simulink library "ConverterLibrary"  (R2026a)
settings: Solver=VariableStepAuto
undefined symbols (not defined in the file or in its folder): DiscIntNeverNeededParam, dspblkCoreblockFVToolHelper, gcbh, gridInverter
libraries: fl_lib x240, nesl_utility x221, ee_lib x208, slpidlib x28, eeGeneralControl x12, simulink x9, eeTransforms x4, simulink_extras x1, eePowerMeasurement x1
(part 25 of 30)

== system ConverterLibrary/Power Converter Plant/Soft-Switching Converters/LLC Converter/LLC Primary Inverter and Resonant Tank/LLC Detailed Model/Inverter/Primary Inverter ==
  G1 : Inport
  G2 : Inport  Port=2
  G3 : Inport  Port=3
  G4 : Inport  Port=4
  Full Bridge with Thermal : Subsystem  VariantControl=FullBridgewithThermal
      settings: PortSchema="{\"entries\":[{\"content\":{\"sides\":[{\"content\":{\"connectorIds\":[\"LConn1\",\"LConn2\"]},\"type\":\"ConnectorPlacement.EquallySpacedRectSide\",\"uuid\":\"27c41940-d662-4779-afdd-48b642f77411\"},{\"content\":{\"connectorIds\":[\"RConn1\",\"RConn2\"],\"side\":\"RIGHT\"},\"type\":\"ConnectorPlacement.EquallySpacedRectSide\",\"uuid\":\"b0072b01-add1-4b0f-b94e-e1b6c9886b0e\"},{\"content\":{\"connectorIds\":[\"In1\",\"In2\",\"In3\",\"In4\"],\"side\":\"TOP\"},\"type\":\"ConnectorPlacement.EquallySpacedRectSide\",\"uuid\":\"c43bed80-422d-49db-9596-8b38d5c3e411\"},{\"content\":{\"side\":\"BOTTOM\"},\"type\":\"ConnectorPlacement.EquallySpacedRectSide\",\"uuid\":\"01f06046-f57e-45b0-bca5-368a5a543f97\"}]},\"type\":\"ConnectorPlacement.EquallySpacedConnector\",\"uuid\":\"2fcb5370-6bd7-4702-bf87-ebedbb7e376c\"}],\"packageUris\":[\"http://schema.mathworks.com/mf0/Connector/R2020b\"],\"version\":\"1.0\"}"
  Half Bridge with Thermal : Subsystem  VariantControl=HalfBridgewithThermal
      settings: PortSchema="{\"entries\":[{\"content\":{\"sides\":[{\"content\":{\"connectorIds\":[\"LConn1\",\"LConn2\"]},\"type\":\"ConnectorPlacement.EquallySpacedRectSide\",\"uuid\":\"27c41940-d662-4779-afdd-48b642f77411\"},{\"content\":{\"connectorIds\":[\"RConn1\",\"RConn2\"],\"side\":\"RIGHT\"},\"type\":\"ConnectorPlacement.EquallySpacedRectSide\",\"uuid\":\"b0072b01-add1-4b0f-b94e-e1b6c9886b0e\"},{\"content\":{\"connectorIds\":[\"In1\",\"In2\",\"In3\",\"In4\"],\"side\":\"TOP\"},\"type\":\"ConnectorPlacement.EquallySpacedRectSide\",\"uuid\":\"c43bed80-422d-49db-9596-8b38d5c3e411\"},{\"content\":{\"side\":\"BOTTOM\"},\"type\":\"ConnectorPlacement.EquallySpacedRectSide\",\"uuid\":\"01f06046-f57e-45b0-bca5-368a5a543f97\"}]},\"type\":\"ConnectorPlacement.EquallySpacedConnector\",\"uuid\":\"2fcb5370-6bd7-4702-bf87-ebedbb7e376c\"}],\"packageUris\":[\"http://schema.mathworks.com/mf0/Connector/R2020b\"],\"version\":\"1.0\"}"
  Ideal Switch Full Bridge : Subsystem  VariantControl=FullBridgewithoutThermal
      settings: PortSchema="{\"entries\":[{\"content\":{\"sides\":[{\"content\":{\"connectorIds\":[\"LConn1\",\"LConn2\"]},\"type\":\"ConnectorPlacement.EquallySpacedRectSide\",\"uuid\":\"27c41940-d662-4779-afdd-48b642f77411\"},{\"content\":{\"connectorIds\":[\"RConn1\",\"RConn2\"],\"side\":\"RIGHT\"},\"type\":\"ConnectorPlacement.EquallySpacedRectSide\",\"uuid\":\"b0072b01-add1-4b0f-b94e-e1b6c9886b0e\"},{\"content\":{\"connectorIds\":[\"In1\",\"In2\",\"In3\",\"In4\"],\"side\":\"TOP\"},\"type\":\"ConnectorPlacement.EquallySpacedRectSide\",\"uuid\":\"c43bed80-422d-49db-9596-8b38d5c3e411\"},{\"content\":{\"side\":\"BOTTOM\"},\"type\":\"ConnectorPlacement.EquallySpacedRectSide\",\"uuid\":\"01f06046-f57e-45b0-bca5-368a5a543f97\"}]},\"type\":\"ConnectorPlacement.EquallySpacedConnector\",\"uuid\":\"2fcb5370-6bd7-4702-bf87-ebedbb7e376c\"}],\"packageUris\":[\"http://schema.mathworks.com/mf0/Connector/R2020b\"],\"version\":\"1.0\"}"
  Ideal Switch Half Bridge : Subsystem  VariantControl=HalfBridgewithoutThermal
      settings: PortSchema="{\"entries\":[{\"content\":{\"sides\":[{\"content\":{\"connectorIds\":[\"LConn1\",\"LConn2\"]},\"type\":\"ConnectorPlacement.EquallySpacedRectSide\",\"uuid\":\"27c41940-d662-4779-afdd-48b642f77411\"},{\"content\":{\"connectorIds\":[\"RConn1\",\"RConn2\"],\"side\":\"RIGHT\"},\"type\":\"ConnectorPlacement.EquallySpacedRectSide\",\"uuid\":\"b0072b01-add1-4b0f-b94e-e1b6c9886b0e\"},{\"content\":{\"connectorIds\":[\"In1\",\"In2\",\"In3\",\"In4\"],\"side\":\"TOP\"},\"type\":\"ConnectorPlacement.EquallySpacedRectSide\",\"uuid\":\"c43bed80-422d-49db-9596-8b38d5c3e411\"},{\"content\":{\"side\":\"BOTTOM\"},\"type\":\"ConnectorPlacement.EquallySpacedRectSide\",\"uuid\":\"01f06046-f57e-45b0-bca5-368a5a543f97\"}]},\"type\":\"ConnectorPlacement.EquallySpacedConnector\",\"uuid\":\"2fcb5370-6bd7-4702-bf87-ebedbb7e376c\"}],\"packageUris\":[\"http://schema.mathworks.com/mf0/Connector/R2020b\"],\"version\":\"1.0\"}"
  P1 : PMIOPort  Side=Left
  N1 : PMIOPort  Port=2  Side=Left
  P2 : PMIOPort  Port=3  Side=Right
  N2 : PMIOPort  Port=4  Side=Right

== system ConverterLibrary/Power Converter Plant/Soft-Switching Converters/LLC Converter/LLC Primary Inverter and Resonant Tank/LLC Detailed Model/Inverter/Vin ==
  PS-Simulink Converter : nesl_utility/PS-Simulink Converter  PhysicalDomain=network_engine_domain  SubClassName=ps_output  LeftPortType=input  RightPortType=output  PseudoPeriodic=off  Frequencies=[]  VectorFormat=inherit  Unit=inherit  AffineConversion=off
  Voltage Sensor : fl_lib/Electrical/Electrical Sensors/Voltage Sensor
  + : PMIOPort  Side=Left
  - : PMIOPort  Port=2  Side=Right
  V : Outport
  wires:
  PS-Simulink Converter/1 -> V/1
  connections:
  PS-Simulink Converter/LConn1 -- Voltage Sensor/RConn1
  Voltage Sensor/LConn1 -- +/RConn1
  Voltage Sensor/RConn2 -- -/RConn1

== system ConverterLibrary/Power Converter Plant/Soft-Switching Converters/LLC Converter/LLC Primary Inverter and Resonant Tank/LLC Detailed Model/Resonant Tank/Ip ==
  Current Sensor : fl_lib/Electrical/Electrical Sensors/Current Sensor
  PS-Simulink Converter : nesl_utility/PS-Simulink Converter  PhysicalDomain=network_engine_domain  SubClassName=ps_output  LeftPortType=input  RightPortType=output  PseudoPeriodic=off  Frequencies=[]  VectorFormat=inherit  Unit=inherit  AffineConversion=off
  + : PMIOPort  Side=Left
  - : PMIOPort  Port=2  Side=Right
  I : Outport
  wires:
  PS-Simulink Converter/1 -> I/1
  connections:
  Current Sensor/RConn1 -- PS-Simulink Converter/LConn1
  +/RConn1 -- Current Sensor/LConn1
  Current Sensor/RConn2 -- -/RConn1

== system ConverterLibrary/Power Converter Plant/Soft-Switching Converters/LLC Converter/LLC Primary Inverter and Resonant Tank/LLC Detailed Model/Resonant Tank/Lr ==
  ExternalInductance : Subsystem  VariantControl=ExternalInductance
  LeakageInductance : Subsystem  VariantControl=LeakageInductance
  P : PMIOPort  Side=Left
  N : PMIOPort  Port=2  Side=Right

== system ConverterLibrary/Power Converter Plant/Soft-Switching Converters/LLC Converter/LLC Primary Inverter and Resonant Tank/LLC Detailed Model/Resonant Tank/Vp ==
  PS-Simulink Converter : nesl_utility/PS-Simulink Converter  PhysicalDomain=network_engine_domain  SubClassName=ps_output  LeftPortType=input  RightPortType=output  PseudoPeriodic=off  Frequencies=[]  VectorFormat=inherit  Unit=inherit  AffineConversion=off
  Voltage Sensor : fl_lib/Electrical/Electrical Sensors/Voltage Sensor
  + : PMIOPort  Side=Left
  - : PMIOPort  Port=2  Side=Right
  V : Outport
  wires:
  PS-Simulink Converter/1 -> V/1
  connections:
  PS-Simulink Converter/LConn1 -- Voltage Sensor/RConn1
  Voltage Sensor/LConn1 -- +/RConn1
  Voltage Sensor/RConn2 -- -/RConn1

== system ConverterLibrary/Power Converter Plant/Soft-Switching Converters/LLC Converter/LLC Primary Inverter and Resonant Tank/LLC Detailed Model/Resonant Tank/Vs ==
  PS-Simulink Converter : nesl_utility/PS-Simulink Converter  PhysicalDomain=network_engine_domain  SubClassName=ps_output  LeftPortType=input  RightPortType=output  PseudoPeriodic=off  Frequencies=[]  VectorFormat=inherit  Unit=inherit  AffineConversion=off
  Voltage Sensor : fl_lib/Electrical/Electrical Sensors/Voltage Sensor
  + : PMIOPort  Side=Left
  - : PMIOPort  Port=2  Side=Right
  V : Outport
  wires:
  PS-Simulink Converter/1 -> V/1
  connections:
  PS-Simulink Converter/LConn1 -- Voltage Sensor/RConn1
  Voltage Sensor/LConn1 -- +/RConn1
  Voltage Sensor/RConn2 -- -/RConn1

== system ConverterLibrary/Power Converter Plant/Soft-Switching Converters/LLC Converter/LLC Primary Inverter and Resonant Tank/LLC Simplified Model/Inverter/Half Bridge Converter ==
  G1 : Inport
  G2 : Inport  Port=2
  Diode1 : fl_lib/Electrical/Electrical Elements/Diode  Vf=VfBody V  Ron=RdBody Ohm  Goff=GdBody 1/Ohm  i_specify=off  i_priority=None  i=0 A  i_nominal_specify=off  i_nominal_value=1  i_nominal_unit=A  v_specify=off  v_priority=None  v=0 V  v_nominal_specify=off  v_nominal_value=1  v_nominal_unit=V
  Diode2 : fl_lib/Electrical/Electrical Elements/Diode  Vf=VfBody V  Ron=RdBody Ohm  Goff=GdBody 1/Ohm  i_specify=off  i_priority=None  i=0 A  i_nominal_specify=off  i_nominal_value=1  i_nominal_unit=A  v_specify=off  v_priority=None  v=0 V  v_nominal_specify=off  v_nominal_value=1  v_nominal_unit=V
  Simulink-PS Converter1 : nesl_utility/Simulink-PS Converter  PhysicalDomain=network_engine_domain  SubClassName=ps_input  LeftPortType=input  RightPortType=output  PseudoPeriodic=off  Frequencies=[]  NoiseDistribution=none  NoiseParameters=[]  Unit=1  AffineConversion=off  FilteringAndDerivatives=provide  SimscapeFilterOrder=1  InputFilterTimeConstant=0.001  UdotUserProvided=0
  Simulink-PS Converter2 : nesl_utility/Simulink-PS Converter  PhysicalDomain=network_engine_domain  SubClassName=ps_input  LeftPortType=input  RightPortType=output  PseudoPeriodic=off  Frequencies=[]  NoiseDistribution=none  NoiseParameters=[]  Unit=1  AffineConversion=off  FilteringAndDerivatives=provide  SimscapeFilterOrder=1  InputFilterTimeConstant=0.001  UdotUserProvided=0
  Switch : fl_lib/Electrical/Electrical Elements/Switch  R_closed=RdsOn Ohm  G_open=GdsOff 1/Ohm  Threshold=Vth  i_specify=off  i_priority=None  i=0 A  i_nominal_specify=off  i_nominal_value=1  i_nominal_unit=A  v_specify=off  v_priority=None  v=0 V  v_nominal_specify=off  v_nominal_value=1  v_nominal_unit=V
  Switch1 : fl_lib/Electrical/Electrical Elements/Switch  R_closed=RdsOn Ohm  G_open=GdsOff 1/Ohm  Threshold=Vth  i_specify=off  i_priority=None  i=0 A  i_nominal_specify=off  i_nominal_value=1  i_nominal_unit=A  v_specify=off  v_priority=None  v=0 V  v_nominal_specify=off  v_nominal_value=1  v_nominal_unit=V
  P1 : PMIOPort  Side=Left
  N1 : PMIOPort  Port=2  Side=Left
  P2 : PMIOPort  Port=3  Side=Right
  N2 : PMIOPort  Port=4  Side=Right
  wires:
  G2/1 -> Simulink-PS Converter2/1
  G1/1 -> Simulink-PS Converter1/1
  connections:
  Simulink-PS Converter1/RConn1 -- Switch/RConn1
  Switch1/RConn1 -- Simulink-PS Converter2/RConn1
  N2/RConn1 -- Diode1/LConn1 -- Switch1/LConn1 -- N1/RConn1
  Diode1/RConn1 -- Switch1/RConn2 -- P2/RConn1 -- Switch/LConn1 -- Diode2/LConn1
  P1/RConn1 -- Diode2/RConn1 -- Switch/RConn2

== system ConverterLibrary/Power Converter Plant/Soft-Switching Converters/LLC Converter/LLC Primary Inverter and Resonant Tank/LLC Simplified Model/Inverter/Iin ==
  Current Sensor : fl_lib/Electrical/Electrical Sensors/Current Sensor
  PS-Simulink Converter : nesl_utility/PS-Simulink Converter  PhysicalDomain=network_engine_domain  SubClassName=ps_output  LeftPortType=input  RightPortType=output  PseudoPeriodic=off  Frequencies=[]  VectorFormat=inherit  Unit=inherit  AffineConversion=off
  + : PMIOPort  Side=Left
  - : PMIOPort  Port=2  Side=Right
  I : Outport
  wires:
  PS-Simulink Converter/1 -> I/1
  connections:
  Current Sensor/RConn1 -- PS-Simulink Converter/LConn1
  +/RConn1 -- Current Sensor/LConn1
  Current Sensor/RConn2 -- -/RConn1

== system ConverterLibrary/Power Converter Plant/Soft-Switching Converters/LLC Converter/LLC Primary Inverter and Resonant Tank/LLC Simplified Model/Inverter/Vin ==
  PS-Simulink Converter : nesl_utility/PS-Simulink Converter  PhysicalDomain=network_engine_domain  SubClassName=ps_output  LeftPortType=input  RightPortType=output  PseudoPeriodic=off  Frequencies=[]  VectorFormat=inherit  Unit=inherit  AffineConversion=off
  Voltage Sensor : fl_lib/Electrical/Electrical Sensors/Voltage Sensor
  + : PMIOPort  Side=Left
  - : PMIOPort  Port=2  Side=Right
  V : Outport
  wires:
  PS-Simulink Converter/1 -> V/1
  connections:
  PS-Simulink Converter/LConn1 -- Voltage Sensor/RConn1
  Voltage Sensor/LConn1 -- +/RConn1
  Voltage Sensor/RConn2 -- -/RConn1

== system ConverterLibrary/Power Converter Plant/Soft-Switching Converters/LLC Converter/LLC Primary Inverter and Resonant Tank/LLC Simplified Model/Resonant Tank/Ip ==
  Current Sensor : fl_lib/Electrical/Electrical Sensors/Current Sensor
  PS-Simulink Converter : nesl_utility/PS-Simulink Converter  PhysicalDomain=network_engine_domain  SubClassName=ps_output  LeftPortType=input  RightPortType=output  PseudoPeriodic=off  Frequencies=[]  VectorFormat=inherit  Unit=inherit  AffineConversion=off
  + : PMIOPort  Side=Left
  - : PMIOPort  Port=2  Side=Right
  I : Outport
  wires:
  PS-Simulink Converter/1 -> I/1
  connections:
  Current Sensor/RConn1 -- PS-Simulink Converter/LConn1
  +/RConn1 -- Current Sensor/LConn1
  Current Sensor/RConn2 -- -/RConn1

== system ConverterLibrary/Power Converter Plant/Soft-Switching Converters/LLC Converter/LLC Primary Inverter and Resonant Tank/LLC Simplified Model/Resonant Tank/Is ==
  Current Sensor : fl_lib/Electrical/Electrical Sensors/Current Sensor
  PS-Simulink Converter : nesl_utility/PS-Simulink Converter  PhysicalDomain=network_engine_domain  SubClassName=ps_output  LeftPortType=input  RightPortType=output  PseudoPeriodic=off  Frequencies=[]  VectorFormat=inherit  Unit=inherit  AffineConversion=off
  + : PMIOPort  Side=Left
  - : PMIOPort  Port=2  Side=Right
  I : Outport
  wires:
  PS-Simulink Converter/1 -> I/1
  connections:
  Current Sensor/RConn1 -- PS-Simulink Converter/LConn1
  +/RConn1 -- Current Sensor/LConn1
  Current Sensor/RConn2 -- -/RConn1

== system ConverterLibrary/Power Converter Plant/Soft-Switching Converters/LLC Converter/LLC Primary Inverter and Resonant Tank/LLC Simplified Model/Resonant Tank/Vp ==
  PS-Simulink Converter : nesl_utility/PS-Simulink Converter  PhysicalDomain=network_engine_domain  SubClassName=ps_output  LeftPortType=input  RightPortType=output  PseudoPeriodic=off  Frequencies=[]  VectorFormat=inherit  Unit=inherit  AffineConversion=off
  Voltage Sensor : fl_lib/Electrical/Electrical Sensors/Voltage Sensor
  + : PMIOPort  Side=Left
  - : PMIOPort  Port=2  Side=Right
  V : Outport
  wires:
  PS-Simulink Converter/1 -> V/1
  connections:
  PS-Simulink Converter/LConn1 -- Voltage Sensor/RConn1
  Voltage Sensor/LConn1 -- +/RConn1
  Voltage Sensor/RConn2 -- -/RConn1

== system ConverterLibrary/Power Converter Plant/Soft-Switching Converters/LLC Converter/LLC Primary Inverter and Resonant Tank/LLC Simplified Model/Resonant Tank/Vs ==
  PS-Simulink Converter : nesl_utility/PS-Simulink Converter  PhysicalDomain=network_engine_domain  SubClassName=ps_output  LeftPortType=input  RightPortType=output  PseudoPeriodic=off  Frequencies=[]  VectorFormat=inherit  Unit=inherit  AffineConversion=off
  Voltage Sensor : fl_lib/Electrical/Electrical Sensors/Voltage Sensor
  + : PMIOPort  Side=Left
  - : PMIOPort  Port=2  Side=Right
  V : Outport
  wires:
  PS-Simulink Converter/1 -> V/1
  connections:
  PS-Simulink Converter/LConn1 -- Voltage Sensor/RConn1
  Voltage Sensor/LConn1 -- +/RConn1
  Voltage Sensor/RConn2 -- -/RConn1

== system ConverterLibrary/Power Converter Plant/Soft-Switching Converters/LLC Converter/Rectifier/Rectifier Bridge/Centre-Tap Ideal Diode/Is ==
  Current Sensor : fl_lib/Electrical/Electrical Sensors/Current Sensor
  PS-Simulink Converter : nesl_utility/PS-Simulink Converter  PhysicalDomain=network_engine_domain  SubClassName=ps_output  LeftPortType=input  RightPortType=output  PseudoPeriodic=off  Frequencies=[]  VectorFormat=inherit  Unit=inherit  AffineConversion=off
  + : PMIOPort  Side=Left
  - : PMIOPort  Port=2  Side=Right
  I : Outport
  wires:
  PS-Simulink Converter/1 -> I/1
  connections:
  Current Sensor/RConn1 -- PS-Simulink Converter/LConn1
  +/RConn1 -- Current Sensor/LConn1
  Current Sensor/RConn2 -- -/RConn1

== system ConverterLibrary/Power Converter Plant/Soft-Switching Converters/LLC Converter/Rectifier/Rectifier Bridge/Centre-Tap Tabulated Diode/Is ==
  Current Sensor : fl_lib/Electrical/Electrical Sensors/Current Sensor
  PS-Simulink Converter : nesl_utility/PS-Simulink Converter  PhysicalDomain=network_engine_domain  SubClassName=ps_output  LeftPortType=input  RightPortType=output  PseudoPeriodic=off  Frequencies=[]  VectorFormat=inherit  Unit=inherit  AffineConversion=off
  + : PMIOPort  Side=Left
  - : PMIOPort  Port=2  Side=Right
  I : Outport
  wires:
  PS-Simulink Converter/1 -> I/1
  connections:
  Current Sensor/RConn1 -- PS-Simulink Converter/LConn1
  +/RConn1 -- Current Sensor/LConn1
  Current Sensor/RConn2 -- -/RConn1

== system ConverterLibrary/Power Converter Plant/Soft-Switching Converters/LLC Converter/Rectifier/Rectifier Bridge/Full Bridge Ideal Diode/Is ==
  Current Sensor : fl_lib/Electrical/Electrical Sensors/Current Sensor
  PS-Simulink Converter : nesl_utility/PS-Simulink Converter  PhysicalDomain=network_engine_domain  SubClassName=ps_output  LeftPortType=input  RightPortType=output  PseudoPeriodic=off  Frequencies=[]  VectorFormat=inherit  Unit=inherit  AffineConversion=off
  + : PMIOPort  Side=Left
  - : PMIOPort  Port=2  Side=Right
  I : Outport
  wires:
  PS-Simulink Converter/1 -> I/1
  connections:
  Current Sensor/RConn1 -- PS-Simulink Converter/LConn1
  +/RConn1 -- Current Sensor/LConn1
  Current Sensor/RConn2 -- -/RConn1

== system ConverterLibrary/Power Converter Plant/Soft-Switching Converters/LLC Converter/Rectifier/Rectifier Bridge/Full Bridge Tabulated Diode/Is ==
  Current Sensor : fl_lib/Electrical/Electrical Sensors/Current Sensor
  PS-Simulink Converter : nesl_utility/PS-Simulink Converter  PhysicalDomain=network_engine_domain  SubClassName=ps_output  LeftPortType=input  RightPortType=output  PseudoPeriodic=off  Frequencies=[]  VectorFormat=inherit  Unit=inherit  AffineConversion=off
  + : PMIOPort  Side=Left
  - : PMIOPort  Port=2  Side=Right
  I : Outport
  wires:
  PS-Simulink Converter/1 -> I/1
  connections:
  Current Sensor/RConn1 -- PS-Simulink Converter/LConn1
  +/RConn1 -- Current Sensor/LConn1
  Current Sensor/RConn2 -- -/RConn1

== system ConverterLibrary/Controller/Inverter-Based Resources/Grid-Forming Converter Controller/Current Limiting/CurrentLimitingMethod/currentLimitAndVirtual/Current Saturation/Compare ==
  u : Inport
  Compare To Zero : simulink/Logic and Bit Operations/Compare To Zero  relop=<=  OutDataTypeStr=boolean
  Data Type Conversion : DataTypeConversion  SaturateOnIntegerOverflow=off  RndMeth=Floor
  Out1 : Outport
  wires:
  Data Type Conversion/1 -> Out1/1
  u/1 -> Compare To Zero/1
  Compare To Zero/1 -> Data Type Conversion/1

== system ConverterLibrary/Controller/Inverter-Based Resources/Grid-Forming Converter Controller/Current Limiting/CurrentLimitingMethod/currentLimitAndVirtual/Current Saturation/If Action Subsystem ==
  Is : Inport
  Isd : Inport  Port=2
  Isq : Inport  Port=3
  maxI : Inport  Port=4
  Action Port : ActionPort
  Divide : Product  Inputs=*/
  Product : Product
  Product1 : Product
  Idmax : Outport
  Iqmax : Outport  Port=2
  wires:
  Product/1 -> Iqmax/1
  Product1/1 -> Idmax/1
  Isq/1 -> Product/2
  Isd/1 -> Product1/1
  Divide/1 -> Product/1, Product1/2
  Is/1 -> Divide/2
  maxI/1 -> Divide/1

== system ConverterLibrary/Controller/Inverter-Based Resources/Grid-Forming Converter Controller/Current Limiting/CurrentLimitingMethod/currentLimitAndVirtual/Current Saturation/If Action Subsystem1 ==
  Action Port : ActionPort
  Constant3 : Constant  Value=0
  Constant4 : Constant  Value=0
  Idmax : Outport
  Iqmax : Outport  Port=2
  wires:
  Constant3/1 -> Idmax/1
  Constant4/1 -> Iqmax/1

== system ConverterLibrary/Controller/Inverter-Based Resources/Grid-Forming Converter Controller/Grid Voltage Reactive Power Support/Modifying Reactive Power Reference/Changing the Power Reference/EstimateIqForReactivePower/Low Voltage Support ==
  Vin : Inport
  Vd : Inport  Port=2
  Gain4 : Gain  Gain=lowVoltageSupportGain
  Saturation1 : Saturate  UpperLimit=1  LowerLimit=-1
  Subtract : Sum  Inputs=+-
  Iqsupport : Outport
  wires:
  Vd/1 -> Subtract/2
  Vin/1 -> Subtract/1
  Saturation1/1 -> Iqsupport/1
  Gain4/1 -> Saturation1/1
  Subtract/1 -> Gain4/1

== system ConverterLibrary/Controller/Inverter-Based Resources/Grid-Forming Converter Controller/Measurement/Frequency Measurement/Frequency Measurement/If Action Subsystem/Frequency estimation ==
  sk : Inport
  sk-1 : Inport  Port=2
  k : Inport  Port=3
  k-1 : Inport  Port=4
  Trigger : TriggerPort  VariantControl=(inherit)  InitialTriggerSignalState=positive
  Add1 : Sum  Inputs=+-  OutDataTypeStr=double  AccumDataTypeStr=double  RndMeth=Convergent
  Add2 : Sum
  Constant : Constant
  Delay : Delay  DelayLength=1
  Delay1 : Delay  DelayLength=1
  Divide : Product  Inputs=*/  RndMeth=Ceiling
  Gain : Gain  Gain=2  ParamDataTypeStr=double  RndMeth=Convergent
  Gain2 : Gain  Gain=0.5
  MATLAB Function : MATLAB Function  TreatAsAtomicUnit=on
  f : Outport
  wires:
  sk-1/1 -> MATLAB Function/2(y2)
  sk/1 -> MATLAB Function/1(y1)
  k-1/1 -> MATLAB Function/4(x2)  "x1"
  k/1 -> MATLAB Function/3(x1)
  Delay/1 -> Add1/2
  Gain2/1 -> f/1
  Add2/1 -> Gain2/1
  Delay1/1 -> Add2/2
  Divide/1 -> Delay1/1, Add2/1
  MATLAB Function/1(x) -> Add1/1, Delay/1  "x1-y1/slope"
  Gain/1 -> Divide/2
  Constant/1 -> Divide/1
  Add1/1 -> Gain/1

== system ConverterLibrary/Controller/Inverter-Based Resources/Grid-Forming Converter Controller/Power Control/ActivePowerControl/vsmControl/Damping Frequency/ConstantFreqReference ==
  fref : Inport
  Constant1 : Constant
  Terminator : Terminator
  fmeas : Outport
  wires:
  fref/1 -> Terminator/1
  Constant1/1 -> fmeas/1

== system ConverterLibrary/Controller/Inverter-Based Resources/Grid-Forming Converter Controller/Power Control/ActivePowerControl/vsmControl/Damping Frequency/WithFrequencyMeasurement ==
  fref : Inport
  fmeas : Outport
  wires:
  fref/1 -> fmeas/1

== system ConverterLibrary/Controller/Non-Isolated DC-DC Converters/Non-Isolated DC-DC Controller/Output Mode/PWMSignal/Half Bridge PWM Generator/Ramp Mode/FixedStep ==
  Tsw : Inport
  Initial Ramp Value : InitialCondition  Value=0
  Overshoot Residual : Sum  Inputs=-+
  Period Reached : RelationalOperator  Operator=>  ZeroCross=off
  Time Ramp : DiscreteIntegrator  ExternalReset=rising  InitialConditionSource=external  SampleTime=Ts  ShowStatePort=on  ICPrevOutput=DiscIntNeverNeededParam  ICPrevScaledInput=DiscIntNeverNeededParam
  Unit Rate : Constant
  S : Outport
  wires:
  Unit Rate/1 -> Time Ramp/1
  Period Reached/1 -> Time Ramp/2
  Time Ramp/1 -> S/1
  Tsw/1 -> Overshoot Residual/1, Period Reached/2
  Time Ramp/State -> Period Reached/1, Overshoot Residual/2
  Overshoot Residual/1 -> Initial Ramp Value/1
  Initial Ramp Value/1 -> Time Ramp/3

== system ConverterLibrary/Controller/Non-Isolated DC-DC Converters/Non-Isolated DC-DC Controller/Output Mode/PWMSignal/Half Bridge PWM Generator/Ramp Mode/VariableStep ==
  Tsw : Inport
  Initial Ramp Value : InitialCondition  Value=0
  Overshoot Residual : Sum  Inputs=-+
  Period Reached : RelationalOperator  Operator=>
  Time Ramp : Integrator  ExternalReset=rising  InitialConditionSource=external  ShowStatePort=on
  Unit Rate : Constant
  S : Outport
  wires:
  Unit Rate/1 -> Time Ramp/1
  Period Reached/1 -> Time Ramp/2
  Time Ramp/1 -> S/1
  Tsw/1 -> Overshoot Residual/1, Period Reached/2
  Time Ramp/State -> Period Reached/1, Overshoot Residual/2
  Overshoot Residual/1 -> Initial Ramp Value/1
  Initial Ramp Value/1 -> Time Ramp/3

== system ConverterLibrary/Controller/Power Factor Correction Converters/Totem-Pole Boost PFC Controller/Output Mode/PWMSignal/Half Bridge PWM Generator/Ramp Mode/FixedStep ==
  Tsw : Inport
  Initial Ramp Value : InitialCondition  Value=0
  Overshoot Residual : Sum  Inputs=-+
  Period Reached : RelationalOperator  Operator=>  ZeroCross=off
  Time Ramp : DiscreteIntegrator  ExternalReset=rising  InitialConditionSource=external  SampleTime=(1e-8)  ShowStatePort=on  ICPrevOutput=DiscIntNeverNeededParam  ICPrevScaledInput=DiscIntNeverNeededParam
  Unit Rate : Constant
  S : Outport
  wires:
  Initial Ramp Value/1 -> Time Ramp/3
  Overshoot Residual/1 -> Initial Ramp Value/1
  Time Ramp/State -> Overshoot Residual/2, Period Reached/1
  Tsw/1 -> Period Reached/2, Overshoot Residual/1
  Time Ramp/1 -> S/1
  Period Reached/1 -> Time Ramp/2
  Unit Rate/1 -> Time Ramp/1

== system ConverterLibrary/Controller/Power Factor Correction Converters/Totem-Pole Boost PFC Controller/Output Mode/PWMSignal/Half Bridge PWM Generator/Ramp Mode/VariableStep ==
  Tsw : Inport
  Initial Ramp Value : InitialCondition  Value=0
  Overshoot Residual : Sum  Inputs=-+
  Period Reached : RelationalOperator  Operator=>
  Time Ramp : Integrator  ExternalReset=rising  InitialConditionSource=external  ShowStatePort=on
  Unit Rate : Constant
  S : Outport
  wires:
  Initial Ramp Value/1 -> Time Ramp/3
  Overshoot Residual/1 -> Initial Ramp Value/1
  Time Ramp/State -> Overshoot Residual/2, Period Reached/1
  Tsw/1 -> Period Reached/2, Overshoot Residual/1
  Time Ramp/1 -> S/1
  Period Reached/1 -> Time Ramp/2
  Unit Rate/1 -> Time Ramp/1

== system ConverterLibrary/Controller/Soft-Switching Converters/CLLC Controller/Gate Signal/CLLC PWM Generator/Primary Gate Signal/Ramp Mode/FixedStep ==
  Tsw : Inport
  Initial Ramp Value : InitialCondition  Value=0
  Overshoot Residual : Sum  Inputs=-+
  Period Reached : RelationalOperator  Operator=>  ZeroCross=off
  Time Ramp : DiscreteIntegrator  ExternalReset=rising  InitialConditionSource=external  SampleTime=(pwmSampleTime)  ShowStatePort=on  ICPrevOutput=DiscIntNeverNeededParam  ICPrevScaledInput=DiscIntNeverNeededParam
  Unit Rate : Constant
  S : Outport
  wires:
  Unit Rate/1 -> Time Ramp/1
  Period Reached/1 -> Time Ramp/2
  Time Ramp/1 -> S/1
  Tsw/1 -> Overshoot Residual/1, Period Reached/2
  Time Ramp/State -> Period Reached/1, Overshoot Residual/2
  Overshoot Residual/1 -> Initial Ramp Value/1
  Initial Ramp Value/1 -> Time Ramp/3

== system ConverterLibrary/Controller/Soft-Switching Converters/CLLC Controller/Gate Signal/CLLC PWM Generator/Primary Gate Signal/Ramp Mode/VariableStep ==
  Tsw : Inport
  Initial Ramp Value : InitialCondition  Value=0
  Overshoot Residual : Sum  Inputs=-+
  Period Reached : RelationalOperator  Operator=>
  Time Ramp : Integrator  ExternalReset=rising  InitialConditionSource=external  ShowStatePort=on
  Unit Rate : Constant
  S : Outport
  wires:
  Unit Rate/1 -> Time Ramp/1
  Period Reached/1 -> Time Ramp/2
  Time Ramp/1 -> S/1
  Tsw/1 -> Overshoot Residual/1, Period Reached/2
  Time Ramp/State -> Period Reached/1, Overshoot Residual/2
  Overshoot Residual/1 -> Initial Ramp Value/1
  Initial Ramp Value/1 -> Time Ramp/3

== system ConverterLibrary/Controller/Soft-Switching Converters/CLLC Controller/Gate Signal/CLLC PWM Generator/Synchronous Rectifier/Region Select/Above Resonance ==
  primaryGates : Inport
  permit : Inport  Port=2
  Action Port : ActionPort
  Unused Primary Gates : Terminator
  Gs : Outport  InitialOutput=0
  wires:
  primaryGates/1 -> Unused Primary Gates/1
  permit/1 -> Gs/1

== system ConverterLibrary/Controller/Soft-Switching Converters/CLLC Controller/Gate Signal/CLLC PWM Generator/Synchronous Rectifier/Region Select/Below Resonance ==
  primaryGates : Inport
  permit : Inport  Port=2
  Action Port : ActionPort
  Rectifier Permit : Logic
  Gs : Outport  InitialOutput=0
  wires:
  primaryGates/1 -> Rectifier Permit/1
  permit/1 -> Rectifier Permit/2
  Rectifier Permit/1 -> Gs/1

== system ConverterLibrary/Controller/Soft-Switching Converters/CLLC Controller/Gate Signal/CLLC PWM Generator/Synchronous Rectifier/Region Select/Within Band ==
  primaryGates : Inport
  permit : Inport  Port=2
  Action Port : ActionPort
  Unused Rectifier Permit : Terminator
  Gs : Outport  InitialOutput=0
  wires:
  permit/1 -> Unused Rectifier Permit/1
  primaryGates/1 -> Gs/1

== system ConverterLibrary/Controller/Soft-Switching Converters/CLLC Controller/Gate Signal/CLLC PWM Generator/Synchronous Rectifier/Turn On Delay/Rectifier Ramp Mode ==
  rate : Inport
  FixedStep : Subsystem  VariantControl=FixedStep
  VariableStep : Subsystem  VariantControl=VariableStep
  S : Outport

== system ConverterLibrary/Power Converter Plant/Power Factor Correction Converters/Totem-Pole Boost PFC Converter/TotemPoleBoostPFCVariant/DetailedModel/SlowLeg/Diode/IdealDiode ==
  G : Inport
  DiodeHigh : ee_lib/Semiconductors & Converters/Diode  PartSpecification="{\"CollectionId\":\"SimscapeElectrical\",\"CollectionVersion\":\"1.0.0\",\"DatasetId\":\"Infineon|IDW80C65D1|simscape.electrical.diode\",\"DisplayName\":\"Infineon:IDW80C65D1\"}"  ModelType=ee.enum.diode.modelType.pwl  TableType=ee.enum.diode.tableType.IfMat  IfMat=[0.0001 0.0001 0.1601 0.6065 1.9426 5.4603 12.2546 21.9425 34.4556 49.1982 64.7538 83.3404;0.3114 0.8503 2.3479 5.2232 9.8335 15.9488 23.5801 32.5233 43.1998 54.3228 66.653 79.8979] % Datasheet derived A  VfMat=[.9, 1.15, 1.25, 1.5, 1.75, 2.17, 2.6, 2.85; .58, .68, .75, 1.1, 1.38, 1.77, 2.27, 2.7] % Parameter not set V  TjVec=[25 175] % Datasheet derived degC  VfVec=[0.3258 0.4465 0.5672 0.6878 0.8085 0.9292 1.0498 1.1705 1.2912 1.4118 1.5325 1.6532] % Datasheet derived V  IfVec=[.1, .2, .5, 1, 2, 4, 7, 10] % Parameter not set A  IrMat=[1e-06, 2e-06, 5e-06, 1e-05, 2.5e-05, 5e-05, .0001; 2e-06, 5e-06, 1e-05, 4e-05, 8e-05, .0002, .0005] % Parameter not set A  VrMat=[10, 100, 200, 250, 300, 325, 350; 10, 70, 160, 220, 270, 300, 320] % Parameter not set V  VrVec=[10, 20, 40, 50, 70, 80, 100] % Parameter not set V  IrVec=[1e-06, 2e-06, 5e-06, 1e-05, 2e-05, 5e-05, .0001] % Parameter not set A  Vf=VfSlow_SI V  Ron=RdSlow_SI Ohm  Goff=GdSlow_SI S  prmExp=ee.enum.diode.expParam.useTwo  I12=[.0137, .545] % Parameter not set A  V12=[.6, .7] % Parameter not set V  RS=0.001 Ohm  Tmeas=298.15 % Parameter not set K  IS=1e-12 % Parameter not set A  ec=1 % Parameter not set  I1=0.0137 % Parameter not set A  V1=0.6 % Parameter not set V  N_series=1 % Parameter not set  N_parallel=1 % Parameter not set  ZenerEnable=false % Parameter not set  Rz=0.3 % Parameter not set Ohm  BV=inf % Parameter not set V  C_param=ee.enum.diode.capParam.fixed  CJ=0 % Parameter not set pF  CJ0=5 % Parameter not set pF  Vvec=[.1, 10, 100] % Parameter not set V  Cvec=[3.5, 1, .4] % Parameter not set pF  VJ=1 % Parameter not set V  Mgrad=0.5 % Parameter not set  FC=0.5 % Parameter not set  Q_param=ee.enum.diode.recoveryParam.off  iRM=-7.15 % Parameter not set A  iF=4 % Parameter not set A  didt=-750 % Parameter not set A/us  trr_factor=3 % Parameter not set  trr=115 % Parameter not set ns  Qrr=150 % Parameter not set nA*s  Vr=-600 % Parameter not set V  Ls=150 % Parameter not set nH  Erec=0.03 % Parameter not set J  TT=50 % Parameter not set ns  tau=100 % Parameter not set ns  T_param=ee.enum.diode.temperatureParam.off  Tdevice=298.15 % Parameter not set K  I1_T2=0.245 % Parameter not set A  V1_T2=0.5 % Parameter not set V  IS_T2=1.25e-7 % Parameter not set A  Tmeas2=125 % Parameter not set degC  XTI_param=ee.enum.diode.xtiParam.pn  XTI=3 % Parameter not set  EG_param=ee.enum.diode.egapParam.material_si  EG=1.11 % Parameter not set eV  dBVdT=0 % Parameter not set V/K  enable_fault_input=simscape.enum.onoff.off  i_specify=off  i_priority=None  i=0 A  i_nominal_specify=off  i_nominal_value=1  i_nominal_unit=A  v_specify=off  v_priority=None  v=0 V  v_nominal_specify=off  v_nominal_value=1  v_nominal_unit=V  v_capacitor_specify=off  v_capacitor_priority=None  v_capacitor=0 V  v_capacitor_nominal_specify=off  v_capacitor_nominal_value=1  v_capacitor_nominal_unit=V  Qj_specify=off  Qj_priority=High  Qj=0 C  Qj_nominal_specify=off  Qj_nominal_value=1  Qj_nominal_unit=C  i_diode_specify=off  i_diode_priority=None  i_diode=0 A  i_diode_nominal_specify=off  i_diode_nominal_value=1  i_diode_nominal_unit=A  v_diode_specify=off  v_diode_priority=None  v_diode=0 V  v_diode_nominal_specify=off  v_diode_nominal_value=1  v_diode_nominal_unit=V  i_capacitor_specify=off  i_capacitor_priority=None  i_capacitor=0 A  i_capacitor_nominal_specify=off  i_capacitor_nominal_value=1  i_capacitor_nominal_unit=A  fidelity_level=ee.enum.diode.fidelity.includeChargeDyn  rec_loss_model=ee.enum.diode.reverseRecoveryModel.fixed  ErecVal=0 % Parameter not set J  scaleWithIandV=true % Parameter not set  ErecMat=zeros(2, 3) % Parameter not set J  ErecMat3D=zeros(2, 3, 2) J  TjrecVec=[298.15, 398.15] % Parameter not set K  IfrecVec=[.1, 1, 10] % Parameter not set A  IrecVal=10 % Parameter not set A  VrecVal=10 % Parameter not set V  VrecVec=[0, 100] V  tFilter=1 / 1000 / 100 % Parameter not set s  thermal_network_parameterization=ee.enum.thermalNetworkTopology.junctionCase  Rth=[0, 10] % Parameter not set K/W  Rth_Cauer=[1, 3, 10] % Parameter not set K/W  Rth_Foster=[.08, .14, .22, .16] % Parameter not set K/W  thermal_mass_parameterization=ee.enum.thermalNetwork.timeconstant  thermal_mass=[0, 1] % Parameter not set J/K  thermal_mass_Cauer=[.1, .3, 1] % Parameter not set J/K  thermal_mass_Foster=[.001, .005, .05, .5] % Parameter not set J/K  thermal_time_constant=[0, 10] % Parameter not set s  thermal_time_constant_Cauer=[1, 3, 10] % Parameter not set s  thermal_time_constant_Foster=[7e-05, .0007, .01, .08] % Parameter not set s  thermal_mass_initial_temperatures=[25, 25] % Parameter not set degC  thermal_mass_initial_temperatures_Cauer=[25, 25, 25] % Parameter not set degC  junction_thermal_mass=0.01 % Parameter not set J/K  Tvec_initial_Foster=[25, 25, 25, 25] % Parameter not set degC  no_thermal_network=0 % Parameter not set  junction_temperature_specify=off  junction_temperature_priority=None  junction_temperature=25 degC  junction_temperature_nominal_specify=off  junction_temperature_nominal_value=1  junction_temperature_nominal_unit=degC
      settings: AttributesFormatString=Infineon:IDW80C65D1
  DiodeLow : ee_lib/Semiconductors & Converters/Diode  ModelType=ee.enum.diode.modelType.pwl  TableType=ee.enum.diode.tableType.IfMat  IfMat=[0.0001 0.0001 0.1601 0.6065 1.9426 5.4603 12.2546 21.9425 34.4556 49.1982 64.7538 83.3404;0.3114 0.8503 2.3479 5.2232 9.8335 15.9488 23.5801 32.5233 43.1998 54.3228 66.653 79.8979] % Datasheet derived A  VfMat=[.9, 1.15, 1.25, 1.5, 1.75, 2.17, 2.6, 2.85; .58, .68, .75, 1.1, 1.38, 1.77, 2.27, 2.7] % Parameter not set V  TjVec=[25 175] % Datasheet derived degC  VfVec=[0.3258 0.4465 0.5672 0.6878 0.8085 0.9292 1.0498 1.1705 1.2912 1.4118 1.5325 1.6532] % Datasheet derived V  IfVec=[.1, .2, .5, 1, 2, 4, 7, 10] % Parameter not set A  IrMat=[1e-06, 2e-06, 5e-06, 1e-05, 2.5e-05, 5e-05, .0001; 2e-06, 5e-06, 1e-05, 4e-05, 8e-05, .0002, .0005] % Parameter not set A  VrMat=[10, 100, 200, 250, 300, 325, 350; 10, 70, 160, 220, 270, 300, 320] % Parameter not set V  VrVec=[10, 20, 40, 50, 70, 80, 100] % Parameter not set V  IrVec=[1e-06, 2e-06, 5e-06, 1e-05, 2e-05, 5e-05, .0001] % Parameter not set A  Vf=VfSlow_SI V  Ron=RdSlow_SI Ohm  Goff=GdSlow_SI S  prmExp=ee.enum.diode.expParam.useTwo  I12=[.0137, .545] % Parameter not set A  V12=[.6, .7] % Parameter not set V  RS=0.001 Ohm  Tmeas=298.15 % Parameter not set K  IS=1e-12 % Parameter not set A  ec=1 % Parameter not set  I1=0.0137 % Parameter not set A  V1=0.6 % Parameter not set V  N_series=1 % Parameter not set  N_parallel=1 % Parameter not set  ZenerEnable=false % Parameter not set  Rz=0.3 % Parameter not set Ohm  BV=inf % Parameter not set V  C_param=ee.enum.diode.capParam.fixed  CJ=0 % Parameter not set pF  CJ0=5 % Parameter not set pF  Vvec=[.1, 10, 100] % Parameter not set V  Cvec=[3.5, 1, .4] % Parameter not set pF  VJ=1 % Parameter not set V  Mgrad=0.5 % Parameter not set  FC=0.5 % Parameter not set  Q_param=ee.enum.diode.recoveryParam.off  iRM=-7.15 % Parameter not set A  iF=4 % Parameter not set A  didt=-750 % Parameter not set A/us  trr_factor=3 % Parameter not set  trr=115 % Parameter not set ns  Qrr=150 % Parameter not set nA*s  Vr=-600 % Parameter not set V  Ls=150 % Parameter not set nH  Erec=0.03 % Parameter not set J  TT=50 % Parameter not set ns  tau=100 % Parameter not set ns  T_param=ee.enum.diode.temperatureParam.off  Tdevice=298.15 % Parameter not set K  I1_T2=0.245 % Parameter not set A  V1_T2=0.5 % Parameter not set V  IS_T2=1.25e-7 % Parameter not set A  Tmeas2=125 % Parameter not set degC  XTI_param=ee.enum.diode.xtiParam.pn  XTI=3 % Parameter not set  EG_param=ee.enum.diode.egapParam.material_si  EG=1.11 % Parameter not set eV  dBVdT=0 % Parameter not set V/K  enable_fault_input=simscape.enum.onoff.off  i_specify=off  i_priority=None  i=0 A  i_nominal_specify=off  i_nominal_value=1  i_nominal_unit=A  v_specify=off  v_priority=None  v=0 V  v_nominal_specify=off  v_nominal_value=1  v_nominal_unit=V  v_capacitor_specify=off  v_capacitor_priority=None  v_capacitor=0 V  v_capacitor_nominal_specify=off  v_capacitor_nominal_value=1  v_capacitor_nominal_unit=V  Qj_specify=off  Qj_priority=High  Qj=0 C  Qj_nominal_specify=off  Qj_nominal_value=1  Qj_nominal_unit=C  i_diode_specify=off  i_diode_priority=None  i_diode=0 A  i_diode_nominal_specify=off  i_diode_nominal_value=1  i_diode_nominal_unit=A  v_diode_specify=off  v_diode_priority=None  v_diode=0 V  v_diode_nominal_specify=off  v_diode_nominal_value=1  v_diode_nominal_unit=V  i_capacitor_specify=off  i_capacitor_priority=None  i_capacitor=0 A  i_capacitor_nominal_specify=off  i_capacitor_nominal_value=1  i_capacitor_nominal_unit=A  fidelity_level=ee.enum.diode.fidelity.includeChargeDyn  rec_loss_model=ee.enum.diode.reverseRecoveryModel.fixed  ErecVal=0 % Parameter not set J  scaleWithIandV=true % Parameter not set  ErecMat=zeros(2, 3) % Parameter not set J  ErecMat3D=zeros(2, 3, 2) J  TjrecVec=[298.15, 398.15] % Parameter not set K  IfrecVec=[.1, 1, 10] % Parameter not set A  IrecVal=10 % Parameter not set A  VrecVal=10 % Parameter not set V  VrecVec=[0, 100] V  tFilter=1 / 1000 / 100 % Parameter not set s  thermal_network_parameterization=ee.enum.thermalNetworkTopology.junctionCase  Rth=[0, 10] % Parameter not set K/W  Rth_Cauer=[1, 3, 10] % Parameter not set K/W  Rth_Foster=[.08, .14, .22, .16] % Parameter not set K/W  thermal_mass_parameterization=ee.enum.thermalNetwork.timeconstant  thermal_mass=[0, 1] % Parameter not set J/K  thermal_mass_Cauer=[.1, .3, 1] % Parameter not set J/K  thermal_mass_Foster=[.001, .005, .05, .5] % Parameter not set J/K  thermal_time_constant=[0, 10] % Parameter not set s  thermal_time_constant_Cauer=[1, 3, 10] % Parameter not set s  thermal_time_constant_Foster=[7e-05, .0007, .01, .08] % Parameter not set s  thermal_mass_initial_temperatures=[25, 25] % Parameter not set degC  thermal_mass_initial_temperatures_Cauer=[25, 25, 25] % Parameter not set degC  junction_thermal_mass=0.01 % Parameter not set J/K  Tvec_initial_Foster=[25, 25, 25, 25] % Parameter not set degC  no_thermal_network=0 % Parameter not set  junction_temperature_specify=off  junction_temperature_priority=None  junction_temperature=25 degC  junction_temperature_nominal_specify=off  junction_temperature_nominal_value=1  junction_temperature_nominal_unit=degC
  Term : Terminator
  DC+ : PMIOPort  Side=Right
  Mid : PMIOPort  Port=2  Side=Left
  DC- : PMIOPort  Port=3  Side=Right
  wires:
  G/1 -> Term/1
  connections:
  Mid/RConn1 -- DiodeHigh/LConn1 -- DiodeLow/RConn1
  DC-/RConn1 -- DiodeLow/LConn1
  DiodeHigh/RConn1 -- DC+/RConn1
